simulink model "mech_sim"  (R2023a)
settings: Solver=VariableStepAuto  StartTime=0.0  StopTime=5  RelTol=1e-3
libraries: fl_lib x15, nesl_utility x6
settings Model: Creator=ahmad  LastModifiedBy=ahmad
settings SimscapeCC: SimscapeLogType=all

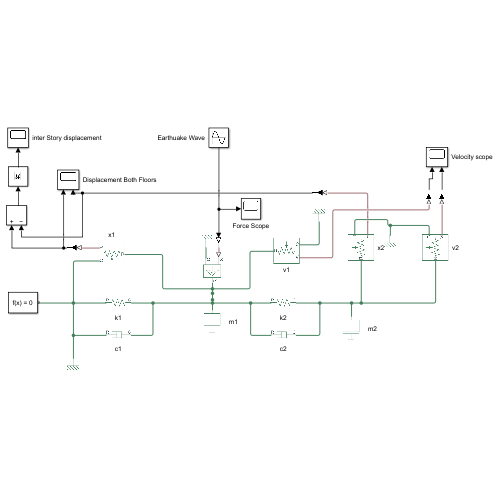
[thumbnail: Simulink's stored preview of the top-level diagram]
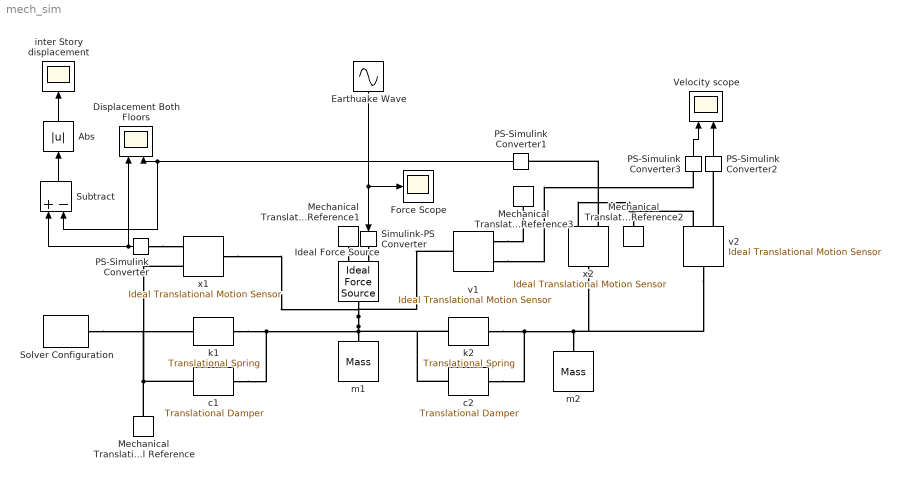
== system mech_sim ==
  Abs : Abs  SaturateOnIntegerOverflow=off
  Displacement Both Floors : Scope  NumInputPorts=2
  Earthuake Wave : Sin  Amplitude=5000  Frequency=8*pi  SampleTime=0
  Force Scope : Scope
  Ideal Force Source : fl_lib/Mechanical/Mechanical Sources/Ideal Force Source
  Mechanical Translational Reference{,1..3} (4 alike) : fl_lib/Mechanical/Translational Elements/Mechanical Translational Reference
  PS-Simulink Converter{,1..3} (4 alike) : nesl_utility/PS-Simulink Converter  PhysicalDomain=network_engine_domain  SubClassName=ps_output  LeftPortType=input  RightPortType=output  PseudoPeriodic=off  Frequencies=[]  VectorFormat=inherit  Unit=inherit  AffineConversion=off
  Simulink-PS Converter : nesl_utility/Simulink-PS Converter  PhysicalDomain=network_engine_domain  SubClassName=ps_input  LeftPortType=input  RightPortType=output  PseudoPeriodic=off  Frequencies=[]  NoiseDistribution=none  NoiseParameters=[]  Unit=1  AffineConversion=off  FilteringAndDerivatives=provide  SimscapeFilterOrder=1  InputFilterTimeConstant=0.001  UdotUserProvided=0
  Solver Configuration : nesl_utility/Solver Configuration  PhysicalDomain=network_engine_domain  SubClassName=solver  LeftPortType=input  RightPortType=generic  Tones=[]  Harmonics=[]  SimulateNoise=off  Profile=off  UseLocalSampling=off  EnableSwitchedLinearOptims=on  FrequencyDomain=off  UseCCode=off  RelTol=0.001  AbsTol=0.001  MinStep=1e-09  ToWorkspace=off  RevertToSquareIcSolve=off  NumHomotopyIterations=100  PhasorMode=off  PhasorModeNumHarmonics=1  ConsistencySolver=NEWTON_XTOL_AFTER_FTOL  IndexReductionMethod=DerivativeReplacement  DoDC=off  ResidualTolerance=1e-09  ConsistencyTolSource=GLOBAL  ConsistencyAbsTol=0.001  ConsistencyRelTol=0.001  ConsistencyTolFactor=0.001  UseLocalSolver=off  LocalSolverChoice=NE_BACKWARD_EULER_ADVANCER  ResolveIndetEquations=on  FunctionEvalNumThread=1  LocalSolverSampleTime=0.001  DoFixedCost=off  MaxNonlinIter=3  MaxModeIter=2  ComputeImpulses=off  ImpulseIterations=2  LinearAlgebra=auto  LinearAlgebraNumThread=0  EquationFormulation=NE_TIME_EF  DelaysMemoryBudget=1024  AutomaticFiltering=on  FilteringTimeConstant=0.001  PartitionStorageMethod=AS_NEEDED  PartitionMemoryBudget=1024  PartitionMethod=ROBUST
  Subtract : Sum  Inputs=+-
  Velocity scope : Scope  NumInputPorts=2
  c1 : fl_lib/Mechanical/Translational Elements/Translational Damper  D=4e6 N*s/m  v_specify=on  v_priority=None  v=0 m/s  v_nominal_specify=off  v_nominal_unit=m/s  v_nominal_value=1  f_specify=off  f_priority=None  f=0 N  f_nominal_specify=off  f_nominal_unit=N  f_nominal_value=1
  c2 : fl_lib/Mechanical/Translational Elements/Translational Damper  D=2e6 N*s/m  v_specify=on  v_priority=None  v=0 m/s  v_nominal_specify=off  v_nominal_unit=m/s  v_nominal_value=1  f_specify=off  f_priority=None  f=0 N  f_nominal_specify=off  f_nominal_unit=N  f_nominal_value=1
  inter Story displacement : Scope
  k1 : fl_lib/Mechanical/Translational Elements/Translational Spring  spr_rate=4e6 N/m  v_specify=off  v_priority=None  v=0 m/s  v_nominal_specify=off  v_nominal_unit=m/s  v_nominal_value=1  f_specify=off  f_priority=None  f=0 N  f_nominal_specify=off  f_nominal_unit=N  f_nominal_value=1  x_specify=on  x_priority=High  x=0 m  x_nominal_specify=off  x_nominal_unit=m  x_nominal_value=1
  k2 : fl_lib/Mechanical/Translational Elements/Translational Spring  spr_rate=2e5 N/m  v_specify=off  v_priority=None  v=0 m/s  v_nominal_specify=off  v_nominal_unit=m/s  v_nominal_value=1  f_specify=off  f_priority=None  f=0 N  f_nominal_specify=off  f_nominal_unit=N  f_nominal_value=1  x_specify=on  x_priority=High  x=0 m  x_nominal_specify=off  x_nominal_unit=m  x_nominal_value=1
  m1 : fl_lib/Mechanical/Translational Elements/Mass  mass=4000 kg  num_ports=foundation.enum.numPorts2.one  v_specify=off  v_priority=High  v=0 m/s  v_nominal_specify=off  v_nominal_unit=m/s  v_nominal_value=1  f_specify=off  f_priority=None  f=0 N  f_nominal_specify=off  f_nominal_unit=N  f_nominal_value=1
  m2 : fl_lib/Mechanical/Translational Elements/Mass  mass=200 kg  num_ports=foundation.enum.numPorts2.one  v_specify=off  v_priority=High  v=0 m/s  v_nominal_specify=off  v_nominal_unit=m/s  v_nominal_value=1  f_specify=off  f_priority=None  f=0 N  f_nominal_specify=off  f_nominal_unit=N  f_nominal_value=1
  v1 : fl_lib/Mechanical/Mechanical Sensors/Ideal Translational Motion Sensor  reference=foundation.enum.MeasurementReference.difference  acceleration_port=false  velocity_port=true  position_port=false  offset=0 m
      settings: InternalSimscapePortConfiguration="{\"Bottom\":[],\"Left\":[{\"id\":\"R\",\"label\":\"R\",\"type\":\"foundation.mechanical.translational.translational\"}],\"Right\":[{\"id\":\"C\",\"label\":\"C\",\"type\":\"foundation.mechanical.translational.translational\"},{\"id\":\"V\",\"label\":\"V\",\"type\":\"output\"}],\"Top\":[]}"
  v2 : fl_lib/Mechanical/Mechanical Sensors/Ideal Translational Motion Sensor  reference=foundation.enum.MeasurementReference.difference  acceleration_port=false  velocity_port=true  position_port=false  offset=0 m
      settings: InternalSimscapePortConfiguration="{\"Bottom\":[],\"Left\":[{\"id\":\"R\",\"label\":\"R\",\"type\":\"foundation.mechanical.translational.translational\"}],\"Right\":[{\"id\":\"C\",\"label\":\"C\",\"type\":\"foundation.mechanical.translational.translational\"},{\"id\":\"V\",\"label\":\"V\",\"type\":\"output\"}],\"Top\":[]}"
  x1 : fl_lib/Mechanical/Mechanical Sensors/Ideal Translational Motion Sensor  reference=foundation.enum.MeasurementReference.difference  acceleration_port=false  velocity_port=false  position_port=true  offset=0 m
      settings: InternalSimscapePortConfiguration="{\"Bottom\":[],\"Left\":[{\"id\":\"R\",\"label\":\"R\",\"type\":\"foundation.mechanical.translational.translational\"}],\"Right\":[{\"id\":\"C\",\"label\":\"C\",\"type\":\"foundation.mechanical.translational.translational\"},{\"id\":\"P\",\"label\":\"P\",\"type\":\"output\"}],\"Top\":[]}"
  x2 : fl_lib/Mechanical/Mechanical Sensors/Ideal Translational Motion Sensor  reference=foundation.enum.MeasurementReference.difference  acceleration_port=false  velocity_port=false  position_port=true  offset=0 m
      settings: InternalSimscapePortConfiguration="{\"Bottom\":[],\"Left\":[{\"id\":\"R\",\"label\":\"R\",\"type\":\"foundation.mechanical.translational.translational\"}],\"Right\":[{\"id\":\"C\",\"label\":\"C\",\"type\":\"foundation.mechanical.translational.translational\"},{\"id\":\"P\",\"label\":\"P\",\"type\":\"output\"}],\"Top\":[]}"
  wires:
  Earthuake Wave/1 -> Force Scope/1, Simulink-PS Converter/1
  PS-Simulink Converter/1 -> Subtract/1, Displacement Both Floors/1
  PS-Simulink Converter1/1 -> Displacement Both Floors/2, Subtract/2
  PS-Simulink Converter2/1 -> Velocity scope/2
  Subtract/1 -> Abs/1
  Abs/1 -> inter Story displacement/1
  PS-Simulink Converter3/1 -> Velocity scope/1
  connections:
  Mechanical Translational Reference/LConn1 -- Solver Configuration/RConn1 -- x1/RConn1 -- k1/LConn1 -- c1/LConn1
  k1/RConn1 -- c1/RConn1 -- v1/LConn1 -- x1/LConn1 -- Ideal Force Source/LConn1 -- m1/LConn1 -- c2/LConn1 -- k2/LConn1
  k2/RConn1 -- c2/RConn1 -- v2/LConn1 -- x2/LConn1 -- m2/LConn1
  Simulink-PS Converter/RConn1 -- Ideal Force Source/RConn1
  Mechanical Translational Reference1/LConn1 -- Ideal Force Source/RConn2
  x2/RConn1 -- v2/RConn1 -- Mechanical Translational Reference2/LConn1
  v1/RConn1 -- Mechanical Translational Reference3/LConn1
  PS-Simulink Converter/LConn1 -- x1/RConn2
  x2/RConn2 -- PS-Simulink Converter1/LConn1
  v1/RConn2 -- PS-Simulink Converter3/LConn1
  v2/RConn2 -- PS-Simulink Converter2/LConn1
